simulink model "PowerSplitGeartrain_Component_harness_model"  (R2023a)
settings: Solver=daessc  StartTime=0.0  StopTime=10.0  RelTol=1e-3
PreLoadFcn:
  | PowerSplitGeartrain_Component_harness_setup
values from neighbouring files (symbols this model uses):
  tireRollingRadius_m = 0.3    [PowerSplitGeartrain_Component_harness_setup.m]
libraries: fl_lib x20, nesl_utility x13, sdl_lib x4
settings Model: Creator=isaacito  LastModifiedBy=isaacito
settings DataIOCC: DSMLogging=off
settings OptimizationCC: ReuseModelBlockBuffer=off
settings SimscapeCC: SimscapeLogType=all  SimscapeLogSimulationStatistics=on  SimscapeLogLimitData=off

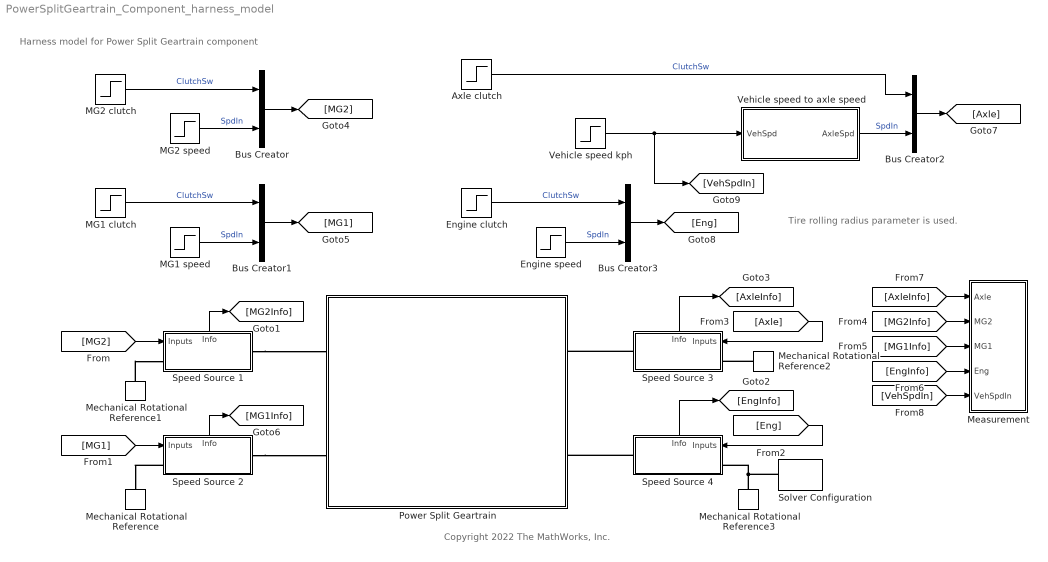
== system PowerSplitGeartrain_Component_harness_model ==
  note: Tire rolling radius parameter is used.
  note: Copyright 2022 The MathWorks, Inc.
  note: Harness model for Power Split Geartrain component
  Axle clutch : Step  Before=1  SampleTime=0
      settings: AttributesFormatString=|
      | Before %<Before>
      | Time %<Time>
      | After %<After>
  Bus Creator{,1..3} (4 alike) : BusCreator  Inputs=2
  Engine clutch : Step  After=0  SampleTime=0
      settings: AttributesFormatString=|
      | Before %<Before>
      | Time %<Time>
      | After %<After>
  Engine speed : Step  After=0  SampleTime=0
      settings: AttributesFormatString=|
      | Before %<Before>
      | Time %<Time>
      | After %<After>
  MG1 clutch : Step  After=0  SampleTime=0
      settings: AttributesFormatString=|
      | Before %<Before>
      | Time %<Time>
      | After %<After>
  MG1 speed : Step  After=0  SampleTime=0
      settings: AttributesFormatString=|
      | Before %<Before>
      | Time %<Time>
      | After %<After>
  MG2 clutch : Step  After=0  SampleTime=0
      settings: AttributesFormatString=|
      | Before %<Before>
      | Time %<Time>
      | After %<After>
  MG2 speed : Step  After=0  SampleTime=0
      settings: AttributesFormatString=|
      | Before %<Before>
      | Time %<Time>
      | After %<After>
  Measurement : Subsystem
  Mechanical Rotational Reference{,1..3} (4 alike) : fl_lib/Mechanical/Rotational Elements/Mechanical Rotational Reference
  Power Split Geartrain : Subsystem  ReferencedSubsystem=PowerSplitGeartrain_refsub_Basic
      settings: PortSchema="{\"entries\":[{\"content\":{\"sides\":[{\"content\":{\"connectorIds\":[\"LConn3\",\"LConn2\"]},\"type\":\"ConnectorPlacement.EquallySpacedRectSide\",\"uuid\":\"39b05f33-5a15-4788-a57f-d6050162e484\"},{\"content\":{\"connectorIds\":[\"LConn1\",\"LConn4\"],\"side\":\"RIGHT\"},\"type\":\"ConnectorPlacement.EquallySpacedRectSide\",\"uuid\":\"22b56448-375b-40fb-9a49-9bd466a0970b\"},{\"content\":{\"side\":\"TOP\"},\"type\":\"ConnectorPlacement.EquallySpacedRectSide\",\"uuid\":\"d8d57956-46e4-4991-901b-1ed920cdc976\"}]},\"type\":\"ConnectorPlacement.EquallySpacedConnector\",\"uuid\":\"bf43f8af-bced-41cd-bdc5-a4c4cabcb371\"}],\"packageUris\":[\"http://schema.mathworks.com/mf0/Connector/R2020b\"],\"version\":\"1.0\"}"
  Solver Configuration : nesl_utility/Solver Configuration  PhysicalDomain=network_engine_domain  SubClassName=solver  LeftPortType=input  RightPortType=generic  Tones=[]  Harmonics=[]  SimulateNoise=off  Profile=off  UseLocalSampling=off  EnableSwitchedLinearOptims=on  FrequencyDomain=off  UseCCode=off  RelTol=0.001  AbsTol=0.001  MinStep=1e-09  ToWorkspace=off  RevertToSquareIcSolve=off  NumHomotopyIterations=100  PhasorMode=off  PhasorModeNumHarmonics=1  ConsistencySolver=NEWTON_XTOL_AFTER_FTOL  IndexReductionMethod=DerivativeReplacement  DoDC=off  ResidualTolerance=1e-09  ConsistencyTolSource=GLOBAL  ConsistencyAbsTol=0.001  ConsistencyRelTol=0.001  ConsistencyTolFactor=0.001  UseLocalSolver=off  LocalSolverChoice=NE_BACKWARD_EULER_ADVANCER  ResolveIndetEquations=on  FunctionEvalNumThread=1  LocalSolverSampleTime=0.001  DoFixedCost=off  MaxNonlinIter=3  MaxModeIter=2  ComputeImpulses=off  ImpulseIterations=2  LinearAlgebra=auto  LinearAlgebraNumThread=0  EquationFormulation=NE_TIME_EF  DelaysMemoryBudget=1024  AutomaticFiltering=on  FilteringTimeConstant=0.001  PartitionStorageMethod=AS_NEEDED  PartitionMemoryBudget=1024  PartitionMethod=ROBUST
  Speed Source 1 : Subsystem
      settings: PortSchema="{\"entries\":[{\"content\":{\"sides\":[{\"content\":{\"connectorIds\":[\"In1\",\"LConn1\"]},\"type\":\"ConnectorPlacement.EquallySpacedRectSide\",\"uuid\":\"92a06674-aaa2-495f-b380-fd1e5a218eb3\"},{\"content\":{\"connectorIds\":[\"RConn1\"],\"side\":\"RIGHT\"},\"type\":\"ConnectorPlacement.EquallySpacedRectSide\",\"uuid\":\"3e9807eb-b215-4ab1-ac02-6574a58f93c0\"},{\"content\":{\"connectorIds\":[\"Out1\"],\"side\":\"TOP\"},\"type\":\"ConnectorPlacement.EquallySpacedRectSide\",\"uuid\":\"937668c8-63b6-43a7-85c7-81bf7d359316\"}]},\"type\":\"ConnectorPlacement.EquallySpacedConnector\",\"uuid\":\"ba9b6e46-9639-4838-8d50-8636a64d3a24\"}],\"packageUris\":[\"http://schema.mathworks.com/mf0/Connector/R2020b\"],\"version\":\"1.0\"}"
  Speed Source 2 : Subsystem
      settings: PortSchema="{\"entries\":[{\"content\":{\"sides\":[{\"content\":{\"connectorIds\":[\"In1\",\"LConn1\"]},\"type\":\"ConnectorPlacement.EquallySpacedRectSide\",\"uuid\":\"92a06674-aaa2-495f-b380-fd1e5a218eb3\"},{\"content\":{\"connectorIds\":[\"RConn1\"],\"side\":\"RIGHT\"},\"type\":\"ConnectorPlacement.EquallySpacedRectSide\",\"uuid\":\"3e9807eb-b215-4ab1-ac02-6574a58f93c0\"},{\"content\":{\"connectorIds\":[\"Out1\"],\"side\":\"TOP\"},\"type\":\"ConnectorPlacement.EquallySpacedRectSide\",\"uuid\":\"937668c8-63b6-43a7-85c7-81bf7d359316\"}]},\"type\":\"ConnectorPlacement.EquallySpacedConnector\",\"uuid\":\"ba9b6e46-9639-4838-8d50-8636a64d3a24\"}],\"packageUris\":[\"http://schema.mathworks.com/mf0/Connector/R2020b\"],\"version\":\"1.0\"}"
  Speed Source 3 : Subsystem
      settings: PortSchema="{\"entries\":[{\"content\":{\"sides\":[{\"content\":{\"connectorIds\":[\"In1\",\"LConn1\"]},\"type\":\"ConnectorPlacement.EquallySpacedRectSide\",\"uuid\":\"92a06674-aaa2-495f-b380-fd1e5a218eb3\"},{\"content\":{\"connectorIds\":[\"RConn1\"],\"side\":\"RIGHT\"},\"type\":\"ConnectorPlacement.EquallySpacedRectSide\",\"uuid\":\"3e9807eb-b215-4ab1-ac02-6574a58f93c0\"},{\"content\":{\"connectorIds\":[\"Out1\"],\"side\":\"TOP\"},\"type\":\"ConnectorPlacement.EquallySpacedRectSide\",\"uuid\":\"937668c8-63b6-43a7-85c7-81bf7d359316\"}]},\"type\":\"ConnectorPlacement.EquallySpacedConnector\",\"uuid\":\"ba9b6e46-9639-4838-8d50-8636a64d3a24\"}],\"packageUris\":[\"http://schema.mathworks.com/mf0/Connector/R2020b\"],\"version\":\"1.0\"}"
  Speed Source 4 : Subsystem
      settings: PortSchema="{\"entries\":[{\"content\":{\"sides\":[{\"content\":{\"connectorIds\":[\"In1\",\"LConn1\"]},\"type\":\"ConnectorPlacement.EquallySpacedRectSide\",\"uuid\":\"92a06674-aaa2-495f-b380-fd1e5a218eb3\"},{\"content\":{\"connectorIds\":[\"RConn1\"],\"side\":\"RIGHT\"},\"type\":\"ConnectorPlacement.EquallySpacedRectSide\",\"uuid\":\"3e9807eb-b215-4ab1-ac02-6574a58f93c0\"},{\"content\":{\"connectorIds\":[\"Out1\"],\"side\":\"TOP\"},\"type\":\"ConnectorPlacement.EquallySpacedRectSide\",\"uuid\":\"937668c8-63b6-43a7-85c7-81bf7d359316\"}]},\"type\":\"ConnectorPlacement.EquallySpacedConnector\",\"uuid\":\"ba9b6e46-9639-4838-8d50-8636a64d3a24\"}],\"packageUris\":[\"http://schema.mathworks.com/mf0/Connector/R2020b\"],\"version\":\"1.0\"}"
  Vehicle speed kph : Step  Before=160  After=160  SampleTime=0
      settings: AttributesFormatString=|
      | Before %<Before>
      | Time %<Time>
      | After %<After>
  Vehicle speed to axle speed : Subsystem
  wires:
  MG2 clutch/1 -> Bus Creator/1  "ClutchSw"
  MG2 speed/1 -> Bus Creator/2  "SpdIn"
  Bus Creator/1 -> [MG2]
  [MG2] -> Speed Source 1/1(Inputs)
  MG1 clutch/1 -> Bus Creator1/1  "ClutchSw"
  MG1 speed/1 -> Bus Creator1/2  "SpdIn"
  Bus Creator1/1 -> [MG1]
  Speed Source 2/1(Info) -> [MG1Info]
  [MG1] -> Speed Source 2/1(Inputs)
  Engine clutch/1 -> Bus Creator3/1  "ClutchSw"
  Engine speed/1 -> Bus Creator3/2  "SpdIn"
  Bus Creator2/1 -> [Axle]
  Bus Creator3/1 -> [Eng]
  Speed Source 4/1(Info) -> [EngInfo]
  Speed Source 3/1(Info) -> [AxleInfo]
  [AxleInfo] -> Measurement/1(Axle)
  [MG2Info] -> Measurement/2(MG2)
  [MG1Info] -> Measurement/3(MG1)
  [EngInfo] -> Measurement/4(Eng)
  Speed Source 1/1(Info) -> [MG2Info]
  [Axle] -> Speed Source 3/1(Inputs)
  [Eng] -> Speed Source 4/1(Inputs)
  Vehicle speed kph/1 -> Vehicle speed to axle speed/1(VehSpd), [VehSpdIn]
  Axle clutch/1 -> Bus Creator2/1  "ClutchSw"
  Vehicle speed to axle speed/1(AxleSpd) -> Bus Creator2/2  "SpdIn"
  [VehSpdIn] -> Measurement/5(VehSpdIn)
  connections:
  Speed Source 1/RConn1 -- Power Split Geartrain/LConn3
  Speed Source 2/RConn1 -- Power Split Geartrain/LConn2
  Speed Source 4/RConn1 -- Power Split Geartrain/LConn4
  Speed Source 3/RConn1 -- Power Split Geartrain/LConn1
  Speed Source 2/LConn1 -- Mechanical Rotational Reference/LConn1
  Mechanical Rotational Reference1/LConn1 -- Speed Source 1/LConn1
  Mechanical Rotational Reference2/LConn1 -- Speed Source 3/LConn1
  Mechanical Rotational Reference3/LConn1 -- Solver Configuration/RConn1 -- Speed Source 4/LConn1

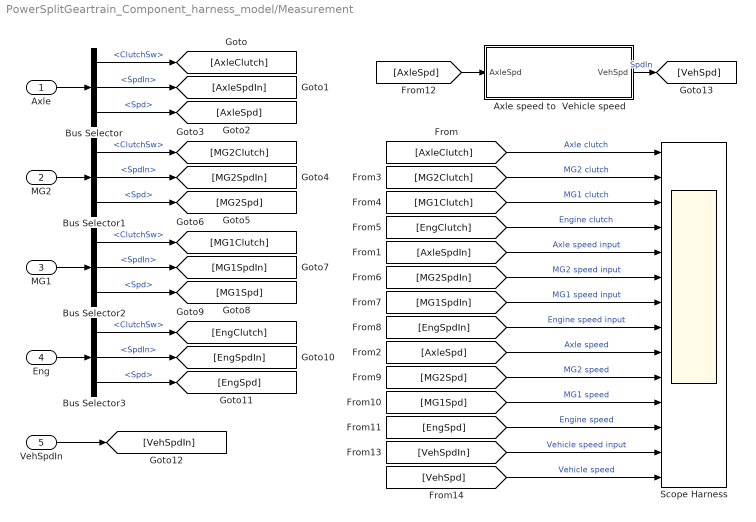
== system PowerSplitGeartrain_Component_harness_model/Measurement ==
  Axle : Inport
  MG2 : Inport  Port=2
  MG1 : Inport  Port=3
  Eng : Inport  Port=4
  VehSpdIn : Inport  Port=5
  Axle speed to  Vehicle speed : Subsystem
  Bus Selector{,1..3} (4 alike) : BusSelector  OutputSignals=ClutchSw,SpdIn,Spd
  Scope Harness : Scope  NumInputPorts=14
  wires:
  Axle/1 -> Bus Selector/1
  Bus Selector/1 -> [AxleClutch]  "<ClutchSw>"
  Bus Selector/2 -> [AxleSpdIn]  "<SpdIn>"
  Bus Selector/3 -> [AxleSpd]  "<Spd>"
  Bus Selector1/3 -> [MG2Spd]  "<Spd>"
  Bus Selector1/2 -> [MG2SpdIn]  "<SpdIn>"
  MG2/1 -> Bus Selector1/1
  Bus Selector1/1 -> [MG2Clutch]  "<ClutchSw>"
  MG1/1 -> Bus Selector2/1
  Bus Selector2/3 -> [MG1Spd]  "<Spd>"
  Bus Selector2/2 -> [MG1SpdIn]  "<SpdIn>"
  Bus Selector2/1 -> [MG1Clutch]  "<ClutchSw>"
  Bus Selector3/2 -> [EngSpdIn]  "<SpdIn>"
  Bus Selector3/3 -> [EngSpd]  "<Spd>"
  Bus Selector3/1 -> [EngClutch]  "<ClutchSw>"
  Eng/1 -> Bus Selector3/1
  [AxleClutch] -> Scope Harness/1  "Axle clutch"
  [MG2Clutch] -> Scope Harness/2  "MG2 clutch"
  [MG1Clutch] -> Scope Harness/3  "MG1 clutch"
  [EngClutch] -> Scope Harness/4  "Engine clutch"
  [AxleSpdIn] -> Scope Harness/5  "Axle speed input"
  [MG2SpdIn] -> Scope Harness/6  "MG2 speed input"
  [MG1SpdIn] -> Scope Harness/7  "MG1 speed input"
  [EngSpdIn] -> Scope Harness/8  "Engine speed input"
  [AxleSpd] -> Scope Harness/9  "Axle speed"
  [MG2Spd] -> Scope Harness/10  "MG2 speed"
  [MG1Spd] -> Scope Harness/11  "MG1 speed"
  [EngSpd] -> Scope Harness/12  "Engine speed"
  [VehSpdIn] -> Scope Harness/13  "Vehicle speed input"
  VehSpdIn/1 -> [VehSpdIn]
  [AxleSpd] -> Axle speed to  Vehicle speed/1(AxleSpd)
  Axle speed to  Vehicle speed/1(VehSpd) -> [VehSpd]  "SpdIn"
  [VehSpd] -> Scope Harness/14  "Vehicle speed"

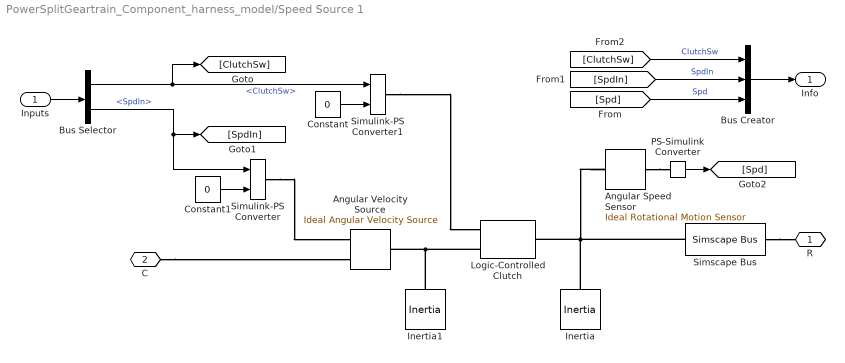
== system PowerSplitGeartrain_Component_harness_model/Speed Source 1 ==
  Inputs : Inport
  Angular Speed Sensor : fl_lib/Mechanical/Mechanical Sensors/Ideal Rotational Motion Sensor  reference=foundation.enum.MeasurementReference.absolute  acceleration_port=false  velocity_port=true  position_port=false  wrap_angle=simscape.enum.onoff.off  offset=0 rad
      settings: InternalSimscapePortConfiguration="{\"Bottom\":[],\"Left\":[{\"id\":\"R\",\"label\":\"R\",\"type\":\"foundation.mechanical.rotational.rotational\"}],\"Right\":[{\"id\":\"W\",\"label\":\"W\",\"type\":\"output\"}],\"Top\":[]}"
  Angular Velocity Source : fl_lib/Mechanical/Mechanical Sources/Ideal Angular Velocity Source
  Bus Creator : BusCreator  Inputs=3
  Bus Selector : BusSelector  OutputSignals=ClutchSw,SpdIn
  Constant : Constant  Value=0
  Constant1 : Constant  Value=0
  Inertia : fl_lib/Mechanical/Rotational Elements/Inertia  inertia=0.01 kg*m^2  num_ports=foundation.enum.numPorts2.one  w_specify=off  w_priority=High  w=0 rad/s  w_nominal_specify=off  w_nominal_unit=rad/s  w_nominal_value=1  t_specify=off  t_priority=None  t=0 N*m  t_nominal_specify=off  t_nominal_unit=N*m  t_nominal_value=1
  Inertia1 : fl_lib/Mechanical/Rotational Elements/Inertia  inertia=0.01 kg*m^2  num_ports=foundation.enum.numPorts2.one  w_specify=on  w_priority=None  w=0 rad/s  w_nominal_specify=off  w_nominal_unit=rad/s  w_nominal_value=1  t_specify=off  t_priority=None  t=0 N*m  t_nominal_specify=off  t_nominal_unit=N*m  t_nominal_value=1
      settings: AttributesFormatString=Priority: %<w_priority>
  Logic-Controlled Clutch : sdl_lib/Clutches/Logic-Controlled Clutch  transition_model=sdl.enum.transitionModel.instant  transition_time_constant=0.1 s  t_friction=5000 kN*m  t_locked=5000 kN*m  w_tol=0.1 rpm  initial_state_locked=sdl.enum.initial_lock.unlocked
      settings: InternalSimscapePortConfiguration="{\"Bottom\":[],\"Left\":[{\"id\":\"E\",\"label\":\"E\",\"type\":\"input\"},{\"id\":\"B\",\"label\":\"B\",\"type\":\"foundation.mechanical.rotational.rotational\"}],\"Right\":[{\"id\":\"F\",\"label\":\"F\",\"type\":\"foundation.mechanical.rotational.rotational\"}],\"Top\":[]}"
  PS-Simulink Converter : nesl_utility/PS-Simulink Converter  PhysicalDomain=network_engine_domain  SubClassName=ps_output  LeftPortType=input  RightPortType=output  PseudoPeriodic=off  Frequencies=[]  VectorFormat=inherit  Unit=rpm  AffineConversion=off
  Simscape Bus : SimscapeBus  HierarchyStrings=AngSpd  ConnectionType=Bus: Bus_Rotational
      settings: AttributesFormatString=%<ConnectionType>
  Simulink-PS Converter : nesl_utility/Simulink-PS Converter  PhysicalDomain=network_engine_domain  SubClassName=ps_input  LeftPortType=input  RightPortType=output  PseudoPeriodic=off  Frequencies=[]  NoiseDistribution=none  NoiseParameters=[]  Unit=rpm  AffineConversion=off  FilteringAndDerivatives=provide  SimscapeFilterOrder=1  InputFilterTimeConstant=0.001  UdotUserProvided=1
  Simulink-PS Converter1 : nesl_utility/Simulink-PS Converter  PhysicalDomain=network_engine_domain  SubClassName=ps_input  LeftPortType=input  RightPortType=output  PseudoPeriodic=off  Frequencies=[]  NoiseDistribution=none  NoiseParameters=[]  Unit=1  AffineConversion=off  FilteringAndDerivatives=provide  SimscapeFilterOrder=1  InputFilterTimeConstant=0.001  UdotUserProvided=1
      settings: AttributesFormatString=|
      | %<Unit>
      | Derivative: %<FilteringAndDerivatives>
  R : PMIOPort  Side=Right
  C : PMIOPort  Port=2  Side=Left
  Info : Outport
  wires:
  Inputs/1 -> Bus Selector/1
  Bus Selector/1 -> Simulink-PS Converter1/1, [ClutchSw]  "<ClutchSw>"
  Bus Selector/2 -> [SpdIn], Simulink-PS Converter/1  "<SpdIn>"
  PS-Simulink Converter/1 -> [Spd]
  Constant/1 -> Simulink-PS Converter1/2
  Constant1/1 -> Simulink-PS Converter/2
  [ClutchSw] -> Bus Creator/1  "ClutchSw"
  [SpdIn] -> Bus Creator/2  "SpdIn"
  [Spd] -> Bus Creator/3  "Spd"
  Bus Creator/1 -> Info/1
  connections:
  Simulink-PS Converter/RConn1 -- Angular Velocity Source/RConn1
  Logic-Controlled Clutch/LConn2 -- Inertia1/LConn1 -- Angular Velocity Source/LConn1
  Simulink-PS Converter1/RConn1 -- Logic-Controlled Clutch/LConn1
  Angular Speed Sensor/LConn1 -- Logic-Controlled Clutch/RConn1 -- Inertia/LConn1 -- Simscape Bus/LConn1
  Angular Speed Sensor/RConn1 -- PS-Simulink Converter/LConn1
  Simscape Bus/RConn1 -- R/RConn1
  C/RConn1 -- Angular Velocity Source/RConn2

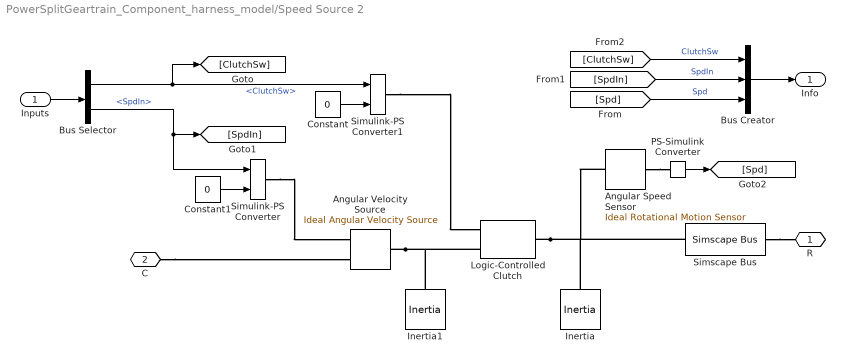
== system PowerSplitGeartrain_Component_harness_model/Speed Source 2 ==
  Inputs : Inport
  Angular Speed Sensor : fl_lib/Mechanical/Mechanical Sensors/Ideal Rotational Motion Sensor  reference=foundation.enum.MeasurementReference.absolute  acceleration_port=false  velocity_port=true  position_port=false  wrap_angle=simscape.enum.onoff.off  offset=0 rad
      settings: InternalSimscapePortConfiguration="{\"Bottom\":[],\"Left\":[{\"id\":\"R\",\"label\":\"R\",\"type\":\"foundation.mechanical.rotational.rotational\"}],\"Right\":[{\"id\":\"W\",\"label\":\"W\",\"type\":\"output\"}],\"Top\":[]}"
  Angular Velocity Source : fl_lib/Mechanical/Mechanical Sources/Ideal Angular Velocity Source
  Bus Creator : BusCreator  Inputs=3
  Bus Selector : BusSelector  OutputSignals=ClutchSw,SpdIn
  Constant : Constant  Value=0
  Constant1 : Constant  Value=0
  Inertia : fl_lib/Mechanical/Rotational Elements/Inertia  inertia=0.01 kg*m^2  num_ports=foundation.enum.numPorts2.one  w_specify=off  w_priority=High  w=0 rad/s  w_nominal_specify=off  w_nominal_unit=rad/s  w_nominal_value=1  t_specify=off  t_priority=None  t=0 N*m  t_nominal_specify=off  t_nominal_unit=N*m  t_nominal_value=1
  Inertia1 : fl_lib/Mechanical/Rotational Elements/Inertia  inertia=0.01 kg*m^2  num_ports=foundation.enum.numPorts2.one  w_specify=on  w_priority=None  w=0 rad/s  w_nominal_specify=off  w_nominal_unit=rad/s  w_nominal_value=1  t_specify=off  t_priority=None  t=0 N*m  t_nominal_specify=off  t_nominal_unit=N*m  t_nominal_value=1
      settings: AttributesFormatString=Priority: %<w_priority>
  Logic-Controlled Clutch : sdl_lib/Clutches/Logic-Controlled Clutch  transition_model=sdl.enum.transitionModel.instant  transition_time_constant=0.1 s  t_friction=5000 kN*m  t_locked=5000 kN*m  w_tol=0.1 rpm  initial_state_locked=sdl.enum.initial_lock.unlocked
      settings: InternalSimscapePortConfiguration="{\"Bottom\":[],\"Left\":[{\"id\":\"E\",\"label\":\"E\",\"type\":\"input\"},{\"id\":\"B\",\"label\":\"B\",\"type\":\"foundation.mechanical.rotational.rotational\"}],\"Right\":[{\"id\":\"F\",\"label\":\"F\",\"type\":\"foundation.mechanical.rotational.rotational\"}],\"Top\":[]}"
  PS-Simulink Converter : nesl_utility/PS-Simulink Converter  PhysicalDomain=network_engine_domain  SubClassName=ps_output  LeftPortType=input  RightPortType=output  PseudoPeriodic=off  Frequencies=[]  VectorFormat=inherit  Unit=rpm  AffineConversion=off
  Simscape Bus : SimscapeBus  HierarchyStrings=AngSpd  ConnectionType=Bus: Bus_Rotational
      settings: AttributesFormatString=%<ConnectionType>
  Simulink-PS Converter : nesl_utility/Simulink-PS Converter  PhysicalDomain=network_engine_domain  SubClassName=ps_input  LeftPortType=input  RightPortType=output  PseudoPeriodic=off  Frequencies=[]  NoiseDistribution=none  NoiseParameters=[]  Unit=rpm  AffineConversion=off  FilteringAndDerivatives=provide  SimscapeFilterOrder=1  InputFilterTimeConstant=0.001  UdotUserProvided=1
  Simulink-PS Converter1 : nesl_utility/Simulink-PS Converter  PhysicalDomain=network_engine_domain  SubClassName=ps_input  LeftPortType=input  RightPortType=output  PseudoPeriodic=off  Frequencies=[]  NoiseDistribution=none  NoiseParameters=[]  Unit=1  AffineConversion=off  FilteringAndDerivatives=provide  SimscapeFilterOrder=1  InputFilterTimeConstant=0.001  UdotUserProvided=1
      settings: AttributesFormatString=|
      | %<Unit>
      | Derivative: %<FilteringAndDerivatives>
  R : PMIOPort  Side=Right
  C : PMIOPort  Port=2  Side=Left
  Info : Outport
  wires:
  Inputs/1 -> Bus Selector/1
  Bus Selector/1 -> Simulink-PS Converter1/1, [ClutchSw]  "<ClutchSw>"
  Bus Selector/2 -> [SpdIn], Simulink-PS Converter/1  "<SpdIn>"
  PS-Simulink Converter/1 -> [Spd]
  Constant/1 -> Simulink-PS Converter1/2
  Constant1/1 -> Simulink-PS Converter/2
  [ClutchSw] -> Bus Creator/1  "ClutchSw"
  [SpdIn] -> Bus Creator/2  "SpdIn"
  [Spd] -> Bus Creator/3  "Spd"
  Bus Creator/1 -> Info/1
  connections:
  Simulink-PS Converter/RConn1 -- Angular Velocity Source/RConn1
  Angular Velocity Source/LConn1 -- Logic-Controlled Clutch/LConn2 -- Inertia1/LConn1
  Simulink-PS Converter1/RConn1 -- Logic-Controlled Clutch/LConn1
  Logic-Controlled Clutch/RConn1 -- Angular Speed Sensor/LConn1 -- Simscape Bus/LConn1 -- Inertia/LConn1
  Angular Speed Sensor/RConn1 -- PS-Simulink Converter/LConn1
  Simscape Bus/RConn1 -- R/RConn1
  C/RConn1 -- Angular Velocity Source/RConn2

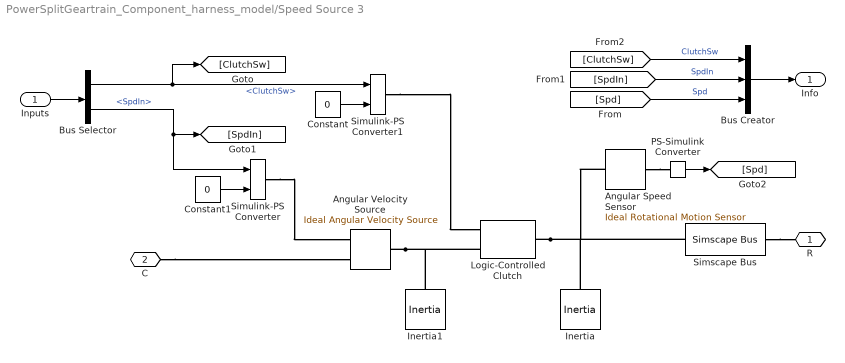
== system PowerSplitGeartrain_Component_harness_model/Speed Source 3 ==
  Inputs : Inport
  Angular Speed Sensor : fl_lib/Mechanical/Mechanical Sensors/Ideal Rotational Motion Sensor  reference=foundation.enum.MeasurementReference.absolute  acceleration_port=false  velocity_port=true  position_port=false  wrap_angle=simscape.enum.onoff.off  offset=0 rad
      settings: InternalSimscapePortConfiguration="{\"Bottom\":[],\"Left\":[{\"id\":\"R\",\"label\":\"R\",\"type\":\"foundation.mechanical.rotational.rotational\"}],\"Right\":[{\"id\":\"W\",\"label\":\"W\",\"type\":\"output\"}],\"Top\":[]}"
  Angular Velocity Source : fl_lib/Mechanical/Mechanical Sources/Ideal Angular Velocity Source
  Bus Creator : BusCreator  Inputs=3
  Bus Selector : BusSelector  OutputSignals=ClutchSw,SpdIn
  Constant : Constant  Value=0
  Constant1 : Constant  Value=0
  Inertia : fl_lib/Mechanical/Rotational Elements/Inertia  inertia=0.01 kg*m^2  num_ports=foundation.enum.numPorts2.one  w_specify=off  w_priority=High  w=0 rad/s  w_nominal_specify=off  w_nominal_unit=rad/s  w_nominal_value=1  t_specify=off  t_priority=None  t=0 N*m  t_nominal_specify=off  t_nominal_unit=N*m  t_nominal_value=1
  Inertia1 : fl_lib/Mechanical/Rotational Elements/Inertia  inertia=0.01 kg*m^2  num_ports=foundation.enum.numPorts2.one  w_specify=on  w_priority=None  w=0 rad/s  w_nominal_specify=off  w_nominal_unit=rad/s  w_nominal_value=1  t_specify=off  t_priority=None  t=0 N*m  t_nominal_specify=off  t_nominal_unit=N*m  t_nominal_value=1
      settings: AttributesFormatString=Priority: %<w_priority>
  Logic-Controlled Clutch : sdl_lib/Clutches/Logic-Controlled Clutch  transition_model=sdl.enum.transitionModel.instant  transition_time_constant=0.1 s  t_friction=5000 kN*m  t_locked=5000 kN*m  w_tol=0.1 rpm  initial_state_locked=sdl.enum.initial_lock.unlocked
      settings: InternalSimscapePortConfiguration="{\"Bottom\":[],\"Left\":[{\"id\":\"E\",\"label\":\"E\",\"type\":\"input\"},{\"id\":\"B\",\"label\":\"B\",\"type\":\"foundation.mechanical.rotational.rotational\"}],\"Right\":[{\"id\":\"F\",\"label\":\"F\",\"type\":\"foundation.mechanical.rotational.rotational\"}],\"Top\":[]}"
  PS-Simulink Converter : nesl_utility/PS-Simulink Converter  PhysicalDomain=network_engine_domain  SubClassName=ps_output  LeftPortType=input  RightPortType=output  PseudoPeriodic=off  Frequencies=[]  VectorFormat=inherit  Unit=rpm  AffineConversion=off
  Simscape Bus : SimscapeBus  HierarchyStrings=AngSpd  ConnectionType=Bus: Bus_Rotational
      settings: AttributesFormatString=%<ConnectionType>
  Simulink-PS Converter : nesl_utility/Simulink-PS Converter  PhysicalDomain=network_engine_domain  SubClassName=ps_input  LeftPortType=input  RightPortType=output  PseudoPeriodic=off  Frequencies=[]  NoiseDistribution=none  NoiseParameters=[]  Unit=rpm  AffineConversion=off  FilteringAndDerivatives=provide  SimscapeFilterOrder=1  InputFilterTimeConstant=0.001  UdotUserProvided=1
  Simulink-PS Converter1 : nesl_utility/Simulink-PS Converter  PhysicalDomain=network_engine_domain  SubClassName=ps_input  LeftPortType=input  RightPortType=output  PseudoPeriodic=off  Frequencies=[]  NoiseDistribution=none  NoiseParameters=[]  Unit=1  AffineConversion=off  FilteringAndDerivatives=provide  SimscapeFilterOrder=1  InputFilterTimeConstant=0.001  UdotUserProvided=1
      settings: AttributesFormatString=|
      | %<Unit>
      | Derivative: %<FilteringAndDerivatives>
  R : PMIOPort  Side=Right
  C : PMIOPort  Port=2  Side=Left
  Info : Outport
  wires:
  Inputs/1 -> Bus Selector/1
  Bus Selector/1 -> Simulink-PS Converter1/1, [ClutchSw]  "<ClutchSw>"
  Bus Selector/2 -> [SpdIn], Simulink-PS Converter/1  "<SpdIn>"
  PS-Simulink Converter/1 -> [Spd]
  Constant/1 -> Simulink-PS Converter1/2
  Constant1/1 -> Simulink-PS Converter/2
  [ClutchSw] -> Bus Creator/1  "ClutchSw"
  [SpdIn] -> Bus Creator/2  "SpdIn"
  [Spd] -> Bus Creator/3  "Spd"
  Bus Creator/1 -> Info/1
  connections:
  Simulink-PS Converter/RConn1 -- Angular Velocity Source/RConn1
  Angular Velocity Source/LConn1 -- Logic-Controlled Clutch/LConn2 -- Inertia1/LConn1
  Simulink-PS Converter1/RConn1 -- Logic-Controlled Clutch/LConn1
  Logic-Controlled Clutch/RConn1 -- Angular Speed Sensor/LConn1 -- Simscape Bus/LConn1 -- Inertia/LConn1
  Angular Speed Sensor/RConn1 -- PS-Simulink Converter/LConn1
  Simscape Bus/RConn1 -- R/RConn1
  C/RConn1 -- Angular Velocity Source/RConn2

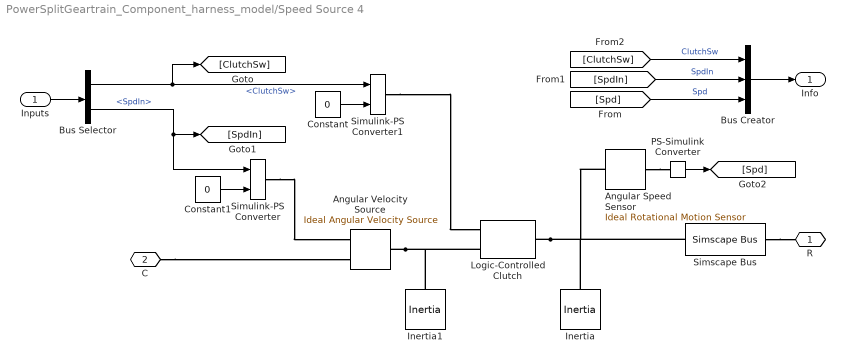
== system PowerSplitGeartrain_Component_harness_model/Speed Source 4 ==
  Inputs : Inport
  Angular Speed Sensor : fl_lib/Mechanical/Mechanical Sensors/Ideal Rotational Motion Sensor  reference=foundation.enum.MeasurementReference.absolute  acceleration_port=false  velocity_port=true  position_port=false  wrap_angle=simscape.enum.onoff.off  offset=0 rad
      settings: InternalSimscapePortConfiguration="{\"Bottom\":[],\"Left\":[{\"id\":\"R\",\"label\":\"R\",\"type\":\"foundation.mechanical.rotational.rotational\"}],\"Right\":[{\"id\":\"W\",\"label\":\"W\",\"type\":\"output\"}],\"Top\":[]}"
  Angular Velocity Source : fl_lib/Mechanical/Mechanical Sources/Ideal Angular Velocity Source
  Bus Creator : BusCreator  Inputs=3
  Bus Selector : BusSelector  OutputSignals=ClutchSw,SpdIn
  Constant : Constant  Value=0
  Constant1 : Constant  Value=0
  Inertia : fl_lib/Mechanical/Rotational Elements/Inertia  inertia=0.01 kg*m^2  num_ports=foundation.enum.numPorts2.one  w_specify=off  w_priority=None  w=0 rad/s  w_nominal_specify=off  w_nominal_unit=rad/s  w_nominal_value=1  t_specify=off  t_priority=None  t=0 N*m  t_nominal_specify=off  t_nominal_unit=N*m  t_nominal_value=1
  Inertia1 : fl_lib/Mechanical/Rotational Elements/Inertia  inertia=0.01 kg*m^2  num_ports=foundation.enum.numPorts2.one  w_specify=on  w_priority=None  w=0 rad/s  w_nominal_specify=off  w_nominal_unit=rad/s  w_nominal_value=1  t_specify=off  t_priority=None  t=0 N*m  t_nominal_specify=off  t_nominal_unit=N*m  t_nominal_value=1
      settings: AttributesFormatString=Priority: %<w_priority>
  Logic-Controlled Clutch : sdl_lib/Clutches/Logic-Controlled Clutch  transition_model=sdl.enum.transitionModel.instant  transition_time_constant=0.1 s  t_friction=5000 kN*m  t_locked=5000 kN*m  w_tol=0.1 rpm  initial_state_locked=sdl.enum.initial_lock.unlocked
      settings: InternalSimscapePortConfiguration="{\"Bottom\":[],\"Left\":[{\"id\":\"E\",\"label\":\"E\",\"type\":\"input\"},{\"id\":\"B\",\"label\":\"B\",\"type\":\"foundation.mechanical.rotational.rotational\"}],\"Right\":[{\"id\":\"F\",\"label\":\"F\",\"type\":\"foundation.mechanical.rotational.rotational\"}],\"Top\":[]}"
  PS-Simulink Converter : nesl_utility/PS-Simulink Converter  PhysicalDomain=network_engine_domain  SubClassName=ps_output  LeftPortType=input  RightPortType=output  PseudoPeriodic=off  Frequencies=[]  VectorFormat=inherit  Unit=rpm  AffineConversion=off
  Simscape Bus : SimscapeBus  HierarchyStrings=AngSpd  ConnectionType=Bus: Bus_Rotational
      settings: AttributesFormatString=%<ConnectionType>
  Simulink-PS Converter : nesl_utility/Simulink-PS Converter  PhysicalDomain=network_engine_domain  SubClassName=ps_input  LeftPortType=input  RightPortType=output  PseudoPeriodic=off  Frequencies=[]  NoiseDistribution=none  NoiseParameters=[]  Unit=rpm  AffineConversion=off  FilteringAndDerivatives=provide  SimscapeFilterOrder=1  InputFilterTimeConstant=0.001  UdotUserProvided=1
  Simulink-PS Converter1 : nesl_utility/Simulink-PS Converter  PhysicalDomain=network_engine_domain  SubClassName=ps_input  LeftPortType=input  RightPortType=output  PseudoPeriodic=off  Frequencies=[]  NoiseDistribution=none  NoiseParameters=[]  Unit=1  AffineConversion=off  FilteringAndDerivatives=provide  SimscapeFilterOrder=1  InputFilterTimeConstant=0.001  UdotUserProvided=1
      settings: AttributesFormatString=|
      | %<Unit>
      | Derivative: %<FilteringAndDerivatives>
  R : PMIOPort  Side=Right
  C : PMIOPort  Port=2  Side=Left
  Info : Outport
  wires:
  Inputs/1 -> Bus Selector/1
  Bus Selector/1 -> Simulink-PS Converter1/1, [ClutchSw]  "<ClutchSw>"
  Bus Selector/2 -> [SpdIn], Simulink-PS Converter/1  "<SpdIn>"
  PS-Simulink Converter/1 -> [Spd]
  Constant/1 -> Simulink-PS Converter1/2
  Constant1/1 -> Simulink-PS Converter/2
  [ClutchSw] -> Bus Creator/1  "ClutchSw"
  [SpdIn] -> Bus Creator/2  "SpdIn"
  [Spd] -> Bus Creator/3  "Spd"
  Bus Creator/1 -> Info/1
  connections:
  Simulink-PS Converter/RConn1 -- Angular Velocity Source/RConn1
  Angular Velocity Source/LConn1 -- Logic-Controlled Clutch/LConn2 -- Inertia1/LConn1
  Simulink-PS Converter1/RConn1 -- Logic-Controlled Clutch/LConn1
  Logic-Controlled Clutch/RConn1 -- Angular Speed Sensor/LConn1 -- Simscape Bus/LConn1 -- Inertia/LConn1
  Angular Speed Sensor/RConn1 -- PS-Simulink Converter/LConn1
  Simscape Bus/RConn1 -- R/RConn1
  C/RConn1 -- Angular Velocity Source/RConn2

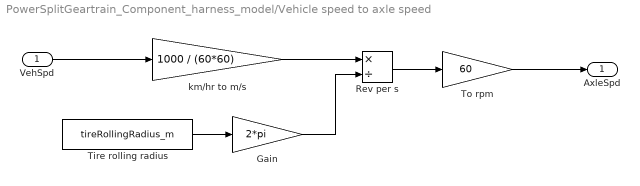
== system PowerSplitGeartrain_Component_harness_model/Vehicle speed to axle speed ==
  VehSpd : Inport  Unit=km/hr
      settings: AttributesFormatString=%<Unit>
  Gain : Gain  Gain=2*pi
  Rev per s : Product  Inputs=*/
  Tire rolling radius : Constant  Value=tireRollingRadius_m
  To rpm : Gain  Gain=60
  km/hr to m/s : Gain  Gain=1000 / (60*60)
  AxleSpd : Outport  Unit=rpm
      settings: AttributesFormatString=%<Unit>
  wires:
  Tire rolling radius/1 -> Gain/1
  km/hr to m/s/1 -> Rev per s/1
  Gain/1 -> Rev per s/2
  Rev per s/1 -> To rpm/1
  To rpm/1 -> AxleSpd/1
  VehSpd/1 -> km/hr to m/s/1

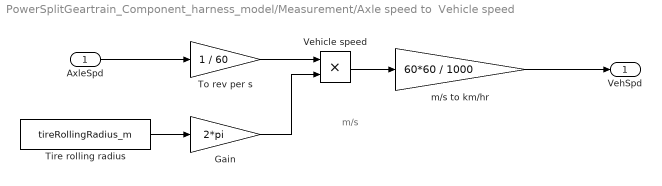
== system PowerSplitGeartrain_Component_harness_model/Measurement/Axle speed to  Vehicle speed ==
  note: m/s
  AxleSpd : Inport  Unit=rpm
      settings: AttributesFormatString=%<Unit>
  Gain : Gain  Gain=2*pi
  Tire rolling radius : Constant  Value=tireRollingRadius_m
  To rev per s : Gain  Gain=1 / 60
  Vehicle speed : Product  Inputs=**
  m/s to km/hr : Gain  Gain=60*60 / 1000
  VehSpd : Outport  Unit=km/hr
      settings: AttributesFormatString=%<Unit>
  wires:
  Tire rolling radius/1 -> Gain/1
  m/s to km/hr/1 -> VehSpd/1
  AxleSpd/1 -> To rev per s/1
  To rev per s/1 -> Vehicle speed/1
  Vehicle speed/1 -> m/s to km/hr/1
  Gain/1 -> Vehicle speed/2
